simulink model "MMC_Rectifier_NLM_2018"  (R2023b)
settings: Solver=ode23t  StartTime=0.0  StopTime=3  RelTol=1e-3
libraries: spsIGBTDiodeLib x216, spsSeriesRLCBranchLib x117, spsVoltageMeasurementLib x110, spsCurrentMeasurementLib x7, slpidlib x6, spsThreePhaseVIMeasurementLib x2, spsGroundLib x1, spsPower3phInstantaneousLib x1, spsThreePhaseProgrammableVoltageSourceLib x1, spsThreePhaseSeriesRLCBranchLib x1, spspowerguiLib x1
(part 2 of 5)

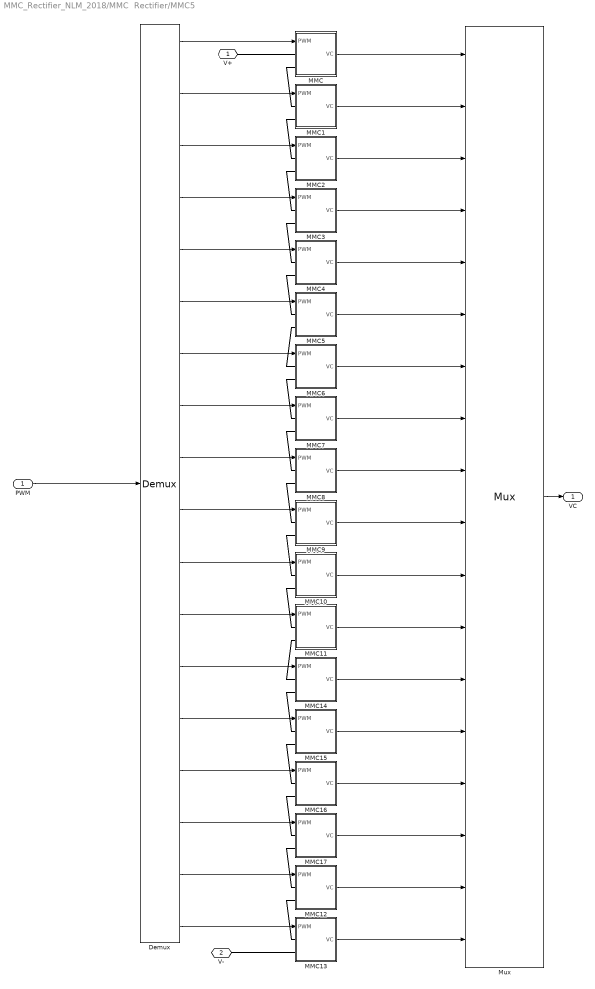
== system MMC_Rectifier_NLM_2018/MMC  Rectifier/MMC5 ==
  PWM : Inport
  Demux : Demux  Outputs=18
  MMC : Subsystem
  MMC1 : Subsystem
  MMC10 : Subsystem
  MMC11 : Subsystem
  MMC12 : Subsystem
  MMC13 : Subsystem
  MMC14 : Subsystem
  MMC15 : Subsystem
  MMC16 : Subsystem
  MMC17 : Subsystem
  MMC2 : Subsystem
  MMC3 : Subsystem
  MMC4 : Subsystem
  MMC5 : Subsystem
  MMC6 : Subsystem
  MMC7 : Subsystem
  MMC8 : Subsystem
  MMC9 : Subsystem
  Mux : Mux  Inputs=18
  V+ : PMIOPort  Side=Left
  V- : PMIOPort  Port=2  Side=Left
  VC : Outport
  wires:
  PWM/1 -> Demux/1
  Demux/18 -> MMC13/1(PWM)
  Demux/17 -> MMC12/1(PWM)
  Demux/16 -> MMC17/1(PWM)
  Demux/15 -> MMC16/1(PWM)
  Demux/14 -> MMC15/1(PWM)
  Demux/13 -> MMC14/1(PWM)
  Demux/12 -> MMC11/1(PWM)
  Demux/11 -> MMC10/1(PWM)
  Demux/10 -> MMC9/1(PWM)
  Demux/9 -> MMC8/1(PWM)
  Demux/8 -> MMC7/1(PWM)
  Demux/7 -> MMC6/1(PWM)
  Demux/6 -> MMC5/1(PWM)
  Demux/5 -> MMC4/1(PWM)
  Demux/4 -> MMC3/1(PWM)
  Demux/3 -> MMC2/1(PWM)
  Demux/2 -> MMC1/1(PWM)
  Demux/1 -> MMC/1(PWM)
  Mux/1 -> VC/1
  MMC13/1(VC) -> Mux/18
  MMC12/1(VC) -> Mux/17
  MMC17/1(VC) -> Mux/16
  MMC16/1(VC) -> Mux/15
  MMC15/1(VC) -> Mux/14
  MMC14/1(VC) -> Mux/13
  MMC11/1(VC) -> Mux/12
  MMC10/1(VC) -> Mux/11
  MMC9/1(VC) -> Mux/10
  MMC8/1(VC) -> Mux/9
  MMC7/1(VC) -> Mux/8
  MMC6/1(VC) -> Mux/7
  MMC5/1(VC) -> Mux/6
  MMC4/1(VC) -> Mux/5
  MMC3/1(VC) -> Mux/4
  MMC2/1(VC) -> Mux/3
  MMC1/1(VC) -> Mux/2
  MMC/1(VC) -> Mux/1
  connections:
  V+/RConn1 -- MMC/LConn1
  V-/RConn1 -- MMC13/LConn2
  MMC6/LConn1 -- MMC5/LConn2
  MMC14/LConn1 -- MMC11/LConn2
  MMC15/LConn2 -- MMC16/LConn1
  MMC17/LConn2 -- MMC12/LConn1
  MMC16/LConn2 -- MMC17/LConn1
  MMC14/LConn2 -- MMC15/LConn1
  MMC12/LConn2 -- MMC13/LConn1
  MMC10/LConn2 -- MMC11/LConn1
  MMC6/LConn2 -- MMC7/LConn1
  MMC7/LConn2 -- MMC8/LConn1
  MMC8/LConn2 -- MMC9/LConn1
  MMC9/LConn2 -- MMC10/LConn1
  MMC3/LConn2 -- MMC4/LConn1
  MMC2/LConn2 -- MMC3/LConn1
  MMC1/LConn2 -- MMC2/LConn1
  MMC/LConn2 -- MMC1/LConn1
  MMC4/LConn2 -- MMC5/LConn1

== system MMC_Rectifier_NLM_2018/坐标变换与锁相环/SOGI1 ==
  v : Inport
  Gain : Gain  Gain=sqrt(2)
  Gain1 : Gain  Gain=100*pi
  Gain2 : Gain  Gain=100*pi
  Integrator : Integrator
  Integrator1 : Integrator
  Sum : Sum  Inputs=|+-
  Sum1 : Sum  Inputs=|+-
  v' : Outport
  qv' : Outport  Port=2
  wires:
  Integrator1/1 -> qv'/1, Sum1/2
  Integrator/1 -> v'/1, Gain2/1, Sum/2
  Gain1/1 -> Integrator/1
  v/1 -> Sum/1
  Sum/1 -> Gain/1
  Sum1/1 -> Gain1/1
  Gain/1 -> Sum1/1
  Gain2/1 -> Integrator1/1

== system MMC_Rectifier_NLM_2018/坐标变换与锁相环/SOGI2 ==
  v : Inport
  Gain : Gain  Gain=sqrt(2)
  Gain1 : Gain  Gain=100*pi
  Gain2 : Gain  Gain=100*pi
  Integrator : Integrator
  Integrator1 : Integrator
  Sum : Sum  Inputs=|+-
  Sum1 : Sum  Inputs=|+-
  v' : Outport
  qv' : Outport  Port=2
  wires:
  Gain2/1 -> Integrator1/1
  Gain/1 -> Sum1/1
  Sum1/1 -> Gain1/1
  Sum/1 -> Gain/1
  v/1 -> Sum/1
  Gain1/1 -> Integrator/1
  Integrator/1 -> Sum/2, Gain2/1, v'/1
  Integrator1/1 -> Sum1/2, qv'/1

== system MMC_Rectifier_NLM_2018/子模块投入个数/Subsystem ==
  VA : Inport
  HLA : Inport  Port=2
  Constant2 : Constant  Value=N/2
  Constant3 : Constant  Value=1400
  Product : Product  Inputs=*/
  Round : Rounding  Operator=round
  Sum : Sum  Inputs=|+-
  Sum1 : Sum  Inputs=|++
  NAP : Outport
  wires:
  VA/1 -> Sum1/1
  HLA/1 -> Sum1/2
  Round/1 -> Sum/2
  Sum1/1 -> Product/1
  Constant2/1 -> Sum/1
  Product/1 -> Round/1
  Constant3/1 -> Product/2
  Sum/1 -> NAP/1

== system MMC_Rectifier_NLM_2018/子模块投入个数/Subsystem1 ==
  VA : Inport
  HLA : Inport  Port=2
  Constant2 : Constant  Value=N/2
  Constant3 : Constant  Value=1400
  Product : Product  Inputs=*/
  Round : Rounding  Operator=round
  Sum : Sum  Inputs=|++
  Sum1 : Sum  Inputs=|+-
  NAL : Outport
  wires:
  Sum/1 -> NAL/1
  Constant3/1 -> Product/2
  Product/1 -> Round/1
  Constant2/1 -> Sum/1
  Sum1/1 -> Product/1
  Round/1 -> Sum/2
  HLA/1 -> Sum1/2
  VA/1 -> Sum1/1

== system MMC_Rectifier_NLM_2018/子模块投入个数/Subsystem2 ==
  VB : Inport
  HLB : Inport  Port=2
  Constant2 : Constant  Value=N/2
  Constant3 : Constant  Value=1400
  Product : Product  Inputs=*/
  Round : Rounding  Operator=round
  Sum : Sum  Inputs=|+-
  Sum1 : Sum  Inputs=|++
  NBP : Outport
  wires:
  VB/1 -> Sum1/1
  HLB/1 -> Sum1/2
  Round/1 -> Sum/2
  Sum1/1 -> Product/1
  Constant2/1 -> Sum/1
  Product/1 -> Round/1
  Constant3/1 -> Product/2
  Sum/1 -> NBP/1

== system MMC_Rectifier_NLM_2018/子模块投入个数/Subsystem3 ==
  VB : Inport
  HLB : Inport  Port=2
  Constant2 : Constant  Value=N/2
  Constant3 : Constant  Value=1400
  Product : Product  Inputs=*/
  Round : Rounding  Operator=round
  Sum : Sum  Inputs=|++
  Sum1 : Sum  Inputs=|+-
  NBL : Outport
  wires:
  Sum/1 -> NBL/1
  Constant3/1 -> Product/2
  Product/1 -> Round/1
  Constant2/1 -> Sum/1
  Sum1/1 -> Product/1
  Round/1 -> Sum/2
  HLB/1 -> Sum1/2
  VB/1 -> Sum1/1

== system MMC_Rectifier_NLM_2018/子模块投入个数/Subsystem4 ==
  VC : Inport
  HLC : Inport  Port=2
  Constant2 : Constant  Value=N/2
  Constant3 : Constant  Value=1400
  Product : Product  Inputs=*/
  Round : Rounding  Operator=round
  Sum : Sum  Inputs=|+-
  Sum1 : Sum  Inputs=|++
  NCP : Outport
  wires:
  VC/1 -> Sum1/1
  HLC/1 -> Sum1/2
  Round/1 -> Sum/2
  Sum1/1 -> Product/1
  Constant2/1 -> Sum/1
  Product/1 -> Round/1
  Constant3/1 -> Product/2
  Sum/1 -> NCP/1

== system MMC_Rectifier_NLM_2018/子模块投入个数/Subsystem5 ==
  VC : Inport
  HLC : Inport  Port=2
  Constant2 : Constant  Value=N/2
  Constant3 : Constant  Value=1400
  Product : Product  Inputs=*/
  Round : Rounding  Operator=round
  Sum : Sum  Inputs=|++
  Sum1 : Sum  Inputs=|+-
  NCL : Outport
  wires:
  Sum/1 -> NCL/1
  Constant3/1 -> Product/2
  Product/1 -> Round/1
  Constant2/1 -> Sum/1
  Sum1/1 -> Product/1
  Round/1 -> Sum/2
  HLC/1 -> Sum1/2
  VC/1 -> Sum1/1

== system MMC_Rectifier_NLM_2018/MMC  Rectifier/MMC/MMC ==
  PWM : Inport
  IGBT/Diode : spsIGBTDiodeLib/IGBT//Diode  Ron=1e-3  Rs=1e5  Cs=inf  Measurements=off
  IGBT/Diode1 : spsIGBTDiodeLib/IGBT//Diode  Ron=1e-3  Rs=1e5  Cs=inf  Measurements=off
  Logical Operator : Logic  Inputs=1  AllPortsSameDT=off  OutDataTypeStr=boolean
  Logical Operator1 : Logic  Operator=NOT  Inputs=1  AllPortsSameDT=off  OutDataTypeStr=boolean
  Series RLC Branch : spsSeriesRLCBranchLib/Series RLC Branch  LConnTagsString=__new0  RConnTagsString=__new0  BranchType=C  Resistance=1  Inductance=1e-3  SetiL0=off  InitialCurrent=0  Capacitance=C0  Setx0=on  InitialVoltage=V0  Measurements=None
  Voltage Measurement : spsVoltageMeasurementLib/Voltage Measurement  PhasorSimulation=off  OutputType=Complex  PSBequivalent=0
  V+ : PMIOPort  Side=Left
  V- : PMIOPort  Port=2  Side=Left
  VC : Outport
  wires:
  PWM/1 -> Logical Operator1/1, Logical Operator/1
  Logical Operator/1 -> IGBT/Diode/1
  Voltage Measurement/1 -> VC/1
  Logical Operator1/1 -> IGBT/Diode1/1
  connections:
  Series RLC Branch/RConn1 -- Voltage Measurement/LConn2 -- V-/RConn1 -- IGBT/Diode1/RConn1
  IGBT/Diode1/LConn1 -- V+/RConn1 -- IGBT/Diode/RConn1
  Series RLC Branch/LConn1 -- Voltage Measurement/LConn1 -- IGBT/Diode/LConn1

== system MMC_Rectifier_NLM_2018/MMC  Rectifier/MMC/MMC1 ==
  PWM : Inport
  IGBT/Diode : spsIGBTDiodeLib/IGBT//Diode  Ron=1e-3  Rs=1e5  Cs=inf  Measurements=off
  IGBT/Diode1 : spsIGBTDiodeLib/IGBT//Diode  Ron=1e-3  Rs=1e5  Cs=inf  Measurements=off
  Logical Operator : Logic  Inputs=1  AllPortsSameDT=off  OutDataTypeStr=boolean
  Logical Operator1 : Logic  Operator=NOT  Inputs=1  AllPortsSameDT=off  OutDataTypeStr=boolean
  Series RLC Branch : spsSeriesRLCBranchLib/Series RLC Branch  LConnTagsString=__new0  RConnTagsString=__new0  BranchType=C  Resistance=1  Inductance=1e-3  SetiL0=off  InitialCurrent=0  Capacitance=C0  Setx0=on  InitialVoltage=V0  Measurements=None
  Voltage Measurement : spsVoltageMeasurementLib/Voltage Measurement  PhasorSimulation=off  OutputType=Complex  PSBequivalent=0
  V+ : PMIOPort  Side=Left
  V- : PMIOPort  Port=2  Side=Left
  VC : Outport
  wires:
  Logical Operator1/1 -> IGBT/Diode1/1
  Voltage Measurement/1 -> VC/1
  Logical Operator/1 -> IGBT/Diode/1
  PWM/1 -> Logical Operator/1, Logical Operator1/1
  connections:
  Voltage Measurement/LConn1 -- Series RLC Branch/LConn1 -- IGBT/Diode/LConn1
  V+/RConn1 -- IGBT/Diode1/LConn1 -- IGBT/Diode/RConn1
  V-/RConn1 -- IGBT/Diode1/RConn1 -- Series RLC Branch/RConn1 -- Voltage Measurement/LConn2

== system MMC_Rectifier_NLM_2018/MMC  Rectifier/MMC/MMC10 ==
  PWM : Inport
  IGBT/Diode : spsIGBTDiodeLib/IGBT//Diode  Ron=1e-3  Rs=1e5  Cs=inf  Measurements=off
  IGBT/Diode1 : spsIGBTDiodeLib/IGBT//Diode  Ron=1e-3  Rs=1e5  Cs=inf  Measurements=off
  Logical Operator : Logic  Inputs=1  AllPortsSameDT=off  OutDataTypeStr=boolean
  Logical Operator1 : Logic  Operator=NOT  Inputs=1  AllPortsSameDT=off  OutDataTypeStr=boolean
  Series RLC Branch : spsSeriesRLCBranchLib/Series RLC Branch  LConnTagsString=__new0  RConnTagsString=__new0  BranchType=C  Resistance=1  Inductance=1e-3  SetiL0=off  InitialCurrent=0  Capacitance=C0  Setx0=on  InitialVoltage=V0  Measurements=None
  Voltage Measurement : spsVoltageMeasurementLib/Voltage Measurement  PhasorSimulation=off  OutputType=Complex  PSBequivalent=0
  V+ : PMIOPort  Side=Left
  V- : PMIOPort  Port=2  Side=Left
  VC : Outport
  wires:
  Logical Operator1/1 -> IGBT/Diode1/1
  Voltage Measurement/1 -> VC/1
  Logical Operator/1 -> IGBT/Diode/1
  PWM/1 -> Logical Operator/1, Logical Operator1/1
  connections:
  Voltage Measurement/LConn1 -- Series RLC Branch/LConn1 -- IGBT/Diode/LConn1
  V+/RConn1 -- IGBT/Diode1/LConn1 -- IGBT/Diode/RConn1
  V-/RConn1 -- IGBT/Diode1/RConn1 -- Series RLC Branch/RConn1 -- Voltage Measurement/LConn2

== system MMC_Rectifier_NLM_2018/MMC  Rectifier/MMC/MMC11 ==
  PWM : Inport
  IGBT/Diode : spsIGBTDiodeLib/IGBT//Diode  Ron=1e-3  Rs=1e5  Cs=inf  Measurements=off
  IGBT/Diode1 : spsIGBTDiodeLib/IGBT//Diode  Ron=1e-3  Rs=1e5  Cs=inf  Measurements=off
  Logical Operator : Logic  Inputs=1  AllPortsSameDT=off  OutDataTypeStr=boolean
  Logical Operator1 : Logic  Operator=NOT  Inputs=1  AllPortsSameDT=off  OutDataTypeStr=boolean
  Series RLC Branch : spsSeriesRLCBranchLib/Series RLC Branch  LConnTagsString=__new0  RConnTagsString=__new0  BranchType=C  Resistance=1  Inductance=1e-3  SetiL0=off  InitialCurrent=0  Capacitance=C0  Setx0=on  InitialVoltage=V0  Measurements=None
  Voltage Measurement : spsVoltageMeasurementLib/Voltage Measurement  PhasorSimulation=off  OutputType=Complex  PSBequivalent=0
  V+ : PMIOPort  Side=Left
  V- : PMIOPort  Port=2  Side=Left
  VC : Outport
  wires:
  PWM/1 -> Logical Operator1/1, Logical Operator/1
  Logical Operator/1 -> IGBT/Diode/1
  Voltage Measurement/1 -> VC/1
  Logical Operator1/1 -> IGBT/Diode1/1
  connections:
  Voltage Measurement/LConn2 -- Series RLC Branch/RConn1 -- IGBT/Diode1/RConn1 -- V-/RConn1
  IGBT/Diode/RConn1 -- IGBT/Diode1/LConn1 -- V+/RConn1
  IGBT/Diode/LConn1 -- Series RLC Branch/LConn1 -- Voltage Measurement/LConn1

== system MMC_Rectifier_NLM_2018/MMC  Rectifier/MMC/MMC12 ==
  PWM : Inport
  IGBT/Diode : spsIGBTDiodeLib/IGBT//Diode  Ron=1e-3  Rs=1e5  Cs=inf  Measurements=off
  IGBT/Diode1 : spsIGBTDiodeLib/IGBT//Diode  Ron=1e-3  Rs=1e5  Cs=inf  Measurements=off
  Logical Operator : Logic  Inputs=1  AllPortsSameDT=off  OutDataTypeStr=boolean
  Logical Operator1 : Logic  Operator=NOT  Inputs=1  AllPortsSameDT=off  OutDataTypeStr=boolean
  Series RLC Branch : spsSeriesRLCBranchLib/Series RLC Branch  LConnTagsString=__new0  RConnTagsString=__new0  BranchType=C  Resistance=1  Inductance=1e-3  SetiL0=off  InitialCurrent=0  Capacitance=C0  Setx0=on  InitialVoltage=V0  Measurements=None
  Voltage Measurement : spsVoltageMeasurementLib/Voltage Measurement  PhasorSimulation=off  OutputType=Complex  PSBequivalent=0
  V+ : PMIOPort  Side=Left
  V- : PMIOPort  Port=2  Side=Left
  VC : Outport
  wires:
  PWM/1 -> Logical Operator1/1, Logical Operator/1
  Logical Operator/1 -> IGBT/Diode/1
  Voltage Measurement/1 -> VC/1
  Logical Operator1/1 -> IGBT/Diode1/1
  connections:
  Voltage Measurement/LConn2 -- Series RLC Branch/RConn1 -- IGBT/Diode1/RConn1 -- V-/RConn1
  IGBT/Diode/RConn1 -- IGBT/Diode1/LConn1 -- V+/RConn1
  IGBT/Diode/LConn1 -- Series RLC Branch/LConn1 -- Voltage Measurement/LConn1

== system MMC_Rectifier_NLM_2018/MMC  Rectifier/MMC/MMC13 ==
  PWM : Inport
  IGBT/Diode : spsIGBTDiodeLib/IGBT//Diode  Ron=1e-3  Rs=1e5  Cs=inf  Measurements=off
  IGBT/Diode1 : spsIGBTDiodeLib/IGBT//Diode  Ron=1e-3  Rs=1e5  Cs=inf  Measurements=off
  Logical Operator : Logic  Inputs=1  AllPortsSameDT=off  OutDataTypeStr=boolean
  Logical Operator1 : Logic  Operator=NOT  Inputs=1  AllPortsSameDT=off  OutDataTypeStr=boolean
  Series RLC Branch : spsSeriesRLCBranchLib/Series RLC Branch  LConnTagsString=__new0  RConnTagsString=__new0  BranchType=C  Resistance=1  Inductance=1e-3  SetiL0=off  InitialCurrent=0  Capacitance=C0  Setx0=on  InitialVoltage=V0  Measurements=None
  Voltage Measurement : spsVoltageMeasurementLib/Voltage Measurement  PhasorSimulation=off  OutputType=Complex  PSBequivalent=0
  V+ : PMIOPort  Side=Left
  V- : PMIOPort  Port=2  Side=Left
  VC : Outport
  wires:
  Logical Operator1/1 -> IGBT/Diode1/1
  Voltage Measurement/1 -> VC/1
  Logical Operator/1 -> IGBT/Diode/1
  PWM/1 -> Logical Operator/1, Logical Operator1/1
  connections:
  Voltage Measurement/LConn1 -- Series RLC Branch/LConn1 -- IGBT/Diode/LConn1
  V+/RConn1 -- IGBT/Diode1/LConn1 -- IGBT/Diode/RConn1
  V-/RConn1 -- IGBT/Diode1/RConn1 -- Series RLC Branch/RConn1 -- Voltage Measurement/LConn2

== system MMC_Rectifier_NLM_2018/MMC  Rectifier/MMC/MMC14 ==
  PWM : Inport
  IGBT/Diode : spsIGBTDiodeLib/IGBT//Diode  Ron=1e-3  Rs=1e5  Cs=inf  Measurements=off
  IGBT/Diode1 : spsIGBTDiodeLib/IGBT//Diode  Ron=1e-3  Rs=1e5  Cs=inf  Measurements=off
  Logical Operator : Logic  Inputs=1  AllPortsSameDT=off  OutDataTypeStr=boolean
  Logical Operator1 : Logic  Operator=NOT  Inputs=1  AllPortsSameDT=off  OutDataTypeStr=boolean
  Series RLC Branch : spsSeriesRLCBranchLib/Series RLC Branch  LConnTagsString=__new0  RConnTagsString=__new0  BranchType=C  Resistance=1  Inductance=1e-3  SetiL0=off  InitialCurrent=0  Capacitance=C0  Setx0=on  InitialVoltage=V0  Measurements=None
  Voltage Measurement : spsVoltageMeasurementLib/Voltage Measurement  PhasorSimulation=off  OutputType=Complex  PSBequivalent=0
  V+ : PMIOPort  Side=Left
  V- : PMIOPort  Port=2  Side=Left
  VC : Outport
  wires:
  PWM/1 -> Logical Operator1/1, Logical Operator/1
  Logical Operator/1 -> IGBT/Diode/1
  Voltage Measurement/1 -> VC/1
  Logical Operator1/1 -> IGBT/Diode1/1
  connections:
  Series RLC Branch/RConn1 -- Voltage Measurement/LConn2 -- V-/RConn1 -- IGBT/Diode1/RConn1
  IGBT/Diode1/LConn1 -- V+/RConn1 -- IGBT/Diode/RConn1
  Series RLC Branch/LConn1 -- Voltage Measurement/LConn1 -- IGBT/Diode/LConn1

== system MMC_Rectifier_NLM_2018/MMC  Rectifier/MMC/MMC15 ==
  PWM : Inport
  IGBT/Diode : spsIGBTDiodeLib/IGBT//Diode  Ron=1e-3  Rs=1e5  Cs=inf  Measurements=off
  IGBT/Diode1 : spsIGBTDiodeLib/IGBT//Diode  Ron=1e-3  Rs=1e5  Cs=inf  Measurements=off
  Logical Operator : Logic  Inputs=1  AllPortsSameDT=off  OutDataTypeStr=boolean
  Logical Operator1 : Logic  Operator=NOT  Inputs=1  AllPortsSameDT=off  OutDataTypeStr=boolean
  Series RLC Branch : spsSeriesRLCBranchLib/Series RLC Branch  LConnTagsString=__new0  RConnTagsString=__new0  BranchType=C  Resistance=1  Inductance=1e-3  SetiL0=off  InitialCurrent=0  Capacitance=C0  Setx0=on  InitialVoltage=V0  Measurements=None
  Voltage Measurement : spsVoltageMeasurementLib/Voltage Measurement  PhasorSimulation=off  OutputType=Complex  PSBequivalent=0
  V+ : PMIOPort  Side=Left
  V- : PMIOPort  Port=2  Side=Left
  VC : Outport
  wires:
  Logical Operator1/1 -> IGBT/Diode1/1
  Voltage Measurement/1 -> VC/1
  Logical Operator/1 -> IGBT/Diode/1
  PWM/1 -> Logical Operator/1, Logical Operator1/1
  connections:
  Voltage Measurement/LConn1 -- Series RLC Branch/LConn1 -- IGBT/Diode/LConn1
  V+/RConn1 -- IGBT/Diode1/LConn1 -- IGBT/Diode/RConn1
  V-/RConn1 -- IGBT/Diode1/RConn1 -- Series RLC Branch/RConn1 -- Voltage Measurement/LConn2

== system MMC_Rectifier_NLM_2018/MMC  Rectifier/MMC/MMC16 ==
  PWM : Inport
  IGBT/Diode : spsIGBTDiodeLib/IGBT//Diode  Ron=1e-3  Rs=1e5  Cs=inf  Measurements=off
  IGBT/Diode1 : spsIGBTDiodeLib/IGBT//Diode  Ron=1e-3  Rs=1e5  Cs=inf  Measurements=off
  Logical Operator : Logic  Inputs=1  AllPortsSameDT=off  OutDataTypeStr=boolean
  Logical Operator1 : Logic  Operator=NOT  Inputs=1  AllPortsSameDT=off  OutDataTypeStr=boolean
  Series RLC Branch : spsSeriesRLCBranchLib/Series RLC Branch  LConnTagsString=__new0  RConnTagsString=__new0  BranchType=C  Resistance=1  Inductance=1e-3  SetiL0=off  InitialCurrent=0  Capacitance=C0  Setx0=on  InitialVoltage=V0  Measurements=None
  Voltage Measurement : spsVoltageMeasurementLib/Voltage Measurement  PhasorSimulation=off  OutputType=Complex  PSBequivalent=0
  V+ : PMIOPort  Side=Left
  V- : PMIOPort  Port=2  Side=Left
  VC : Outport
  wires:
  Logical Operator1/1 -> IGBT/Diode1/1
  Voltage Measurement/1 -> VC/1
  Logical Operator/1 -> IGBT/Diode/1
  PWM/1 -> Logical Operator/1, Logical Operator1/1
  connections:
  Voltage Measurement/LConn1 -- Series RLC Branch/LConn1 -- IGBT/Diode/LConn1
  V+/RConn1 -- IGBT/Diode1/LConn1 -- IGBT/Diode/RConn1
  V-/RConn1 -- IGBT/Diode1/RConn1 -- Series RLC Branch/RConn1 -- Voltage Measurement/LConn2

== system MMC_Rectifier_NLM_2018/MMC  Rectifier/MMC/MMC17 ==
  PWM : Inport
  IGBT/Diode : spsIGBTDiodeLib/IGBT//Diode  Ron=1e-3  Rs=1e5  Cs=inf  Measurements=off
  IGBT/Diode1 : spsIGBTDiodeLib/IGBT//Diode  Ron=1e-3  Rs=1e5  Cs=inf  Measurements=off
  Logical Operator : Logic  Inputs=1  AllPortsSameDT=off  OutDataTypeStr=boolean
  Logical Operator1 : Logic  Operator=NOT  Inputs=1  AllPortsSameDT=off  OutDataTypeStr=boolean
  Series RLC Branch : spsSeriesRLCBranchLib/Series RLC Branch  LConnTagsString=__new0  RConnTagsString=__new0  BranchType=C  Resistance=1  Inductance=1e-3  SetiL0=off  InitialCurrent=0  Capacitance=C0  Setx0=on  InitialVoltage=V0  Measurements=None
  Voltage Measurement : spsVoltageMeasurementLib/Voltage Measurement  PhasorSimulation=off  OutputType=Complex  PSBequivalent=0
  V+ : PMIOPort  Side=Left
  V- : PMIOPort  Port=2  Side=Left
  VC : Outport
  wires:
  PWM/1 -> Logical Operator1/1, Logical Operator/1
  Logical Operator/1 -> IGBT/Diode/1
  Voltage Measurement/1 -> VC/1
  Logical Operator1/1 -> IGBT/Diode1/1
  connections:
  Voltage Measurement/LConn2 -- Series RLC Branch/RConn1 -- IGBT/Diode1/RConn1 -- V-/RConn1
  IGBT/Diode/RConn1 -- IGBT/Diode1/LConn1 -- V+/RConn1
  IGBT/Diode/LConn1 -- Series RLC Branch/LConn1 -- Voltage Measurement/LConn1

== system MMC_Rectifier_NLM_2018/MMC  Rectifier/MMC/MMC2 ==
  PWM : Inport
  IGBT/Diode : spsIGBTDiodeLib/IGBT//Diode  Ron=1e-3  Rs=1e5  Cs=inf  Measurements=off
  IGBT/Diode1 : spsIGBTDiodeLib/IGBT//Diode  Ron=1e-3  Rs=1e5  Cs=inf  Measurements=off
  Logical Operator : Logic  Inputs=1  AllPortsSameDT=off  OutDataTypeStr=boolean
  Logical Operator1 : Logic  Operator=NOT  Inputs=1  AllPortsSameDT=off  OutDataTypeStr=boolean
  Series RLC Branch : spsSeriesRLCBranchLib/Series RLC Branch  LConnTagsString=__new0  RConnTagsString=__new0  BranchType=C  Resistance=1  Inductance=1e-3  SetiL0=off  InitialCurrent=0  Capacitance=C0  Setx0=on  InitialVoltage=V0  Measurements=None
  Voltage Measurement : spsVoltageMeasurementLib/Voltage Measurement  PhasorSimulation=off  OutputType=Complex  PSBequivalent=0
  V+ : PMIOPort  Side=Left
  V- : PMIOPort  Port=2  Side=Left
  VC : Outport
  wires:
  Logical Operator1/1 -> IGBT/Diode1/1
  Voltage Measurement/1 -> VC/1
  Logical Operator/1 -> IGBT/Diode/1
  PWM/1 -> Logical Operator/1, Logical Operator1/1
  connections:
  Voltage Measurement/LConn1 -- Series RLC Branch/LConn1 -- IGBT/Diode/LConn1
  V+/RConn1 -- IGBT/Diode1/LConn1 -- IGBT/Diode/RConn1
  V-/RConn1 -- IGBT/Diode1/RConn1 -- Series RLC Branch/RConn1 -- Voltage Measurement/LConn2

== system MMC_Rectifier_NLM_2018/MMC  Rectifier/MMC/MMC3 ==
  PWM : Inport
  IGBT/Diode : spsIGBTDiodeLib/IGBT//Diode  Ron=1e-3  Rs=1e5  Cs=inf  Measurements=off
  IGBT/Diode1 : spsIGBTDiodeLib/IGBT//Diode  Ron=1e-3  Rs=1e5  Cs=inf  Measurements=off
  Logical Operator : Logic  Inputs=1  AllPortsSameDT=off  OutDataTypeStr=boolean
  Logical Operator1 : Logic  Operator=NOT  Inputs=1  AllPortsSameDT=off  OutDataTypeStr=boolean
  Series RLC Branch : spsSeriesRLCBranchLib/Series RLC Branch  LConnTagsString=__new0  RConnTagsString=__new0  BranchType=C  Resistance=1  Inductance=1e-3  SetiL0=off  InitialCurrent=0  Capacitance=C0  Setx0=on  InitialVoltage=V0  Measurements=None
  Voltage Measurement : spsVoltageMeasurementLib/Voltage Measurement  PhasorSimulation=off  OutputType=Complex  PSBequivalent=0
  V+ : PMIOPort  Side=Left
  V- : PMIOPort  Port=2  Side=Left
  VC : Outport
  wires:
  PWM/1 -> Logical Operator1/1, Logical Operator/1
  Logical Operator/1 -> IGBT/Diode/1
  Voltage Measurement/1 -> VC/1
  Logical Operator1/1 -> IGBT/Diode1/1
  connections:
  Voltage Measurement/LConn2 -- Series RLC Branch/RConn1 -- IGBT/Diode1/RConn1 -- V-/RConn1
  IGBT/Diode/RConn1 -- IGBT/Diode1/LConn1 -- V+/RConn1
  IGBT/Diode/LConn1 -- Series RLC Branch/LConn1 -- Voltage Measurement/LConn1

== system MMC_Rectifier_NLM_2018/MMC  Rectifier/MMC/MMC4 ==
  PWM : Inport
  IGBT/Diode : spsIGBTDiodeLib/IGBT//Diode  Ron=1e-3  Rs=1e5  Cs=inf  Measurements=off
  IGBT/Diode1 : spsIGBTDiodeLib/IGBT//Diode  Ron=1e-3  Rs=1e5  Cs=inf  Measurements=off
  Logical Operator : Logic  Inputs=1  AllPortsSameDT=off  OutDataTypeStr=boolean
  Logical Operator1 : Logic  Operator=NOT  Inputs=1  AllPortsSameDT=off  OutDataTypeStr=boolean
  Series RLC Branch : spsSeriesRLCBranchLib/Series RLC Branch  LConnTagsString=__new0  RConnTagsString=__new0  BranchType=C  Resistance=1  Inductance=1e-3  SetiL0=off  InitialCurrent=0  Capacitance=C0  Setx0=on  InitialVoltage=V0  Measurements=None
  Voltage Measurement : spsVoltageMeasurementLib/Voltage Measurement  PhasorSimulation=off  OutputType=Complex  PSBequivalent=0
  V+ : PMIOPort  Side=Left
  V- : PMIOPort  Port=2  Side=Left
  VC : Outport
  wires:
  PWM/1 -> Logical Operator1/1, Logical Operator/1
  Logical Operator/1 -> IGBT/Diode/1
  Voltage Measurement/1 -> VC/1
  Logical Operator1/1 -> IGBT/Diode1/1
  connections:
  Voltage Measurement/LConn2 -- Series RLC Branch/RConn1 -- IGBT/Diode1/RConn1 -- V-/RConn1
  IGBT/Diode/RConn1 -- IGBT/Diode1/LConn1 -- V+/RConn1
  IGBT/Diode/LConn1 -- Series RLC Branch/LConn1 -- Voltage Measurement/LConn1

== system MMC_Rectifier_NLM_2018/MMC  Rectifier/MMC/MMC5 ==
  PWM : Inport
  IGBT/Diode : spsIGBTDiodeLib/IGBT//Diode  Ron=1e-3  Rs=1e5  Cs=inf  Measurements=off
  IGBT/Diode1 : spsIGBTDiodeLib/IGBT//Diode  Ron=1e-3  Rs=1e5  Cs=inf  Measurements=off
  Logical Operator : Logic  Inputs=1  AllPortsSameDT=off  OutDataTypeStr=boolean
  Logical Operator1 : Logic  Operator=NOT  Inputs=1  AllPortsSameDT=off  OutDataTypeStr=boolean
  Series RLC Branch : spsSeriesRLCBranchLib/Series RLC Branch  LConnTagsString=__new0  RConnTagsString=__new0  BranchType=C  Resistance=1  Inductance=1e-3  SetiL0=off  InitialCurrent=0  Capacitance=C0  Setx0=on  InitialVoltage=V0  Measurements=None
  Voltage Measurement : spsVoltageMeasurementLib/Voltage Measurement  PhasorSimulation=off  OutputType=Complex  PSBequivalent=0
  V+ : PMIOPort  Side=Left
  V- : PMIOPort  Port=2  Side=Left
  VC : Outport
  wires:
  Logical Operator1/1 -> IGBT/Diode1/1
  Voltage Measurement/1 -> VC/1
  Logical Operator/1 -> IGBT/Diode/1
  PWM/1 -> Logical Operator/1, Logical Operator1/1
  connections:
  Voltage Measurement/LConn1 -- Series RLC Branch/LConn1 -- IGBT/Diode/LConn1
  V+/RConn1 -- IGBT/Diode1/LConn1 -- IGBT/Diode/RConn1
  V-/RConn1 -- IGBT/Diode1/RConn1 -- Series RLC Branch/RConn1 -- Voltage Measurement/LConn2

== system MMC_Rectifier_NLM_2018/MMC  Rectifier/MMC/MMC6 ==
  PWM : Inport
  IGBT/Diode : spsIGBTDiodeLib/IGBT//Diode  Ron=1e-3  Rs=1e5  Cs=inf  Measurements=off
  IGBT/Diode1 : spsIGBTDiodeLib/IGBT//Diode  Ron=1e-3  Rs=1e5  Cs=inf  Measurements=off
  Logical Operator : Logic  Inputs=1  AllPortsSameDT=off  OutDataTypeStr=boolean
  Logical Operator1 : Logic  Operator=NOT  Inputs=1  AllPortsSameDT=off  OutDataTypeStr=boolean
  Series RLC Branch : spsSeriesRLCBranchLib/Series RLC Branch  LConnTagsString=__new0  RConnTagsString=__new0  BranchType=C  Resistance=1  Inductance=1e-3  SetiL0=off  InitialCurrent=0  Capacitance=C0  Setx0=on  InitialVoltage=V0  Measurements=None
  Voltage Measurement : spsVoltageMeasurementLib/Voltage Measurement  PhasorSimulation=off  OutputType=Complex  PSBequivalent=0
  V+ : PMIOPort  Side=Left
  V- : PMIOPort  Port=2  Side=Left
  VC : Outport
  wires:
  Logical Operator1/1 -> IGBT/Diode1/1
  Voltage Measurement/1 -> VC/1
  Logical Operator/1 -> IGBT/Diode/1
  PWM/1 -> Logical Operator/1, Logical Operator1/1
  connections:
  IGBT/Diode/LConn1 -- Voltage Measurement/LConn1 -- Series RLC Branch/LConn1
  IGBT/Diode/RConn1 -- V+/RConn1 -- IGBT/Diode1/LConn1
  IGBT/Diode1/RConn1 -- V-/RConn1 -- Voltage Measurement/LConn2 -- Series RLC Branch/RConn1

== system MMC_Rectifier_NLM_2018/MMC  Rectifier/MMC/MMC7 ==
  PWM : Inport
  IGBT/Diode : spsIGBTDiodeLib/IGBT//Diode  Ron=1e-3  Rs=1e5  Cs=inf  Measurements=off
  IGBT/Diode1 : spsIGBTDiodeLib/IGBT//Diode  Ron=1e-3  Rs=1e5  Cs=inf  Measurements=off
  Logical Operator : Logic  Inputs=1  AllPortsSameDT=off  OutDataTypeStr=boolean
  Logical Operator1 : Logic  Operator=NOT  Inputs=1  AllPortsSameDT=off  OutDataTypeStr=boolean
  Series RLC Branch : spsSeriesRLCBranchLib/Series RLC Branch  LConnTagsString=__new0  RConnTagsString=__new0  BranchType=C  Resistance=1  Inductance=1e-3  SetiL0=off  InitialCurrent=0  Capacitance=C0  Setx0=on  InitialVoltage=V0  Measurements=None
  Voltage Measurement : spsVoltageMeasurementLib/Voltage Measurement  PhasorSimulation=off  OutputType=Complex  PSBequivalent=0
  V+ : PMIOPort  Side=Left
  V- : PMIOPort  Port=2  Side=Left
  VC : Outport
  wires:
  PWM/1 -> Logical Operator1/1, Logical Operator/1
  Logical Operator/1 -> IGBT/Diode/1
  Voltage Measurement/1 -> VC/1
  Logical Operator1/1 -> IGBT/Diode1/1
  connections:
  Voltage Measurement/LConn2 -- Series RLC Branch/RConn1 -- IGBT/Diode1/RConn1 -- V-/RConn1
  IGBT/Diode/RConn1 -- IGBT/Diode1/LConn1 -- V+/RConn1
  IGBT/Diode/LConn1 -- Series RLC Branch/LConn1 -- Voltage Measurement/LConn1

== system MMC_Rectifier_NLM_2018/MMC  Rectifier/MMC/MMC8 ==
  PWM : Inport
  IGBT/Diode : spsIGBTDiodeLib/IGBT//Diode  Ron=1e-3  Rs=1e5  Cs=inf  Measurements=off
  IGBT/Diode1 : spsIGBTDiodeLib/IGBT//Diode  Ron=1e-3  Rs=1e5  Cs=inf  Measurements=off
  Logical Operator : Logic  Inputs=1  AllPortsSameDT=off  OutDataTypeStr=boolean
  Logical Operator1 : Logic  Operator=NOT  Inputs=1  AllPortsSameDT=off  OutDataTypeStr=boolean
  Series RLC Branch : spsSeriesRLCBranchLib/Series RLC Branch  LConnTagsString=__new0  RConnTagsString=__new0  BranchType=C  Resistance=1  Inductance=1e-3  SetiL0=off  InitialCurrent=0  Capacitance=C0  Setx0=on  InitialVoltage=V0  Measurements=None
  Voltage Measurement : spsVoltageMeasurementLib/Voltage Measurement  PhasorSimulation=off  OutputType=Complex  PSBequivalent=0
  V+ : PMIOPort  Side=Left
  V- : PMIOPort  Port=2  Side=Left
  VC : Outport
  wires:
  PWM/1 -> Logical Operator1/1, Logical Operator/1
  Logical Operator/1 -> IGBT/Diode/1
  Voltage Measurement/1 -> VC/1
  Logical Operator1/1 -> IGBT/Diode1/1
  connections:
  Voltage Measurement/LConn2 -- Series RLC Branch/RConn1 -- IGBT/Diode1/RConn1 -- V-/RConn1
  IGBT/Diode/RConn1 -- IGBT/Diode1/LConn1 -- V+/RConn1
  IGBT/Diode/LConn1 -- Series RLC Branch/LConn1 -- Voltage Measurement/LConn1

== system MMC_Rectifier_NLM_2018/MMC  Rectifier/MMC/MMC9 ==
  PWM : Inport
  IGBT/Diode : spsIGBTDiodeLib/IGBT//Diode  Ron=1e-3  Rs=1e5  Cs=inf  Measurements=off
  IGBT/Diode1 : spsIGBTDiodeLib/IGBT//Diode  Ron=1e-3  Rs=1e5  Cs=inf  Measurements=off
  Logical Operator : Logic  Inputs=1  AllPortsSameDT=off  OutDataTypeStr=boolean
  Logical Operator1 : Logic  Operator=NOT  Inputs=1  AllPortsSameDT=off  OutDataTypeStr=boolean
  Series RLC Branch : spsSeriesRLCBranchLib/Series RLC Branch  LConnTagsString=__new0  RConnTagsString=__new0  BranchType=C  Resistance=1  Inductance=1e-3  SetiL0=off  InitialCurrent=0  Capacitance=C0  Setx0=on  InitialVoltage=V0  Measurements=None
  Voltage Measurement : spsVoltageMeasurementLib/Voltage Measurement  PhasorSimulation=off  OutputType=Complex  PSBequivalent=0
  V+ : PMIOPort  Side=Left
  V- : PMIOPort  Port=2  Side=Left
  VC : Outport
  wires:
  Logical Operator1/1 -> IGBT/Diode1/1
  Voltage Measurement/1 -> VC/1
  Logical Operator/1 -> IGBT/Diode/1
  PWM/1 -> Logical Operator/1, Logical Operator1/1
  connections:
  Voltage Measurement/LConn1 -- Series RLC Branch/LConn1 -- IGBT/Diode/LConn1
  V+/RConn1 -- IGBT/Diode1/LConn1 -- IGBT/Diode/RConn1
  V-/RConn1 -- IGBT/Diode1/RConn1 -- Series RLC Branch/RConn1 -- Voltage Measurement/LConn2

== system MMC_Rectifier_NLM_2018/MMC  Rectifier/MMC1/MMC ==
  PWM : Inport
  IGBT/Diode : spsIGBTDiodeLib/IGBT//Diode  Ron=1e-3  Rs=1e5  Cs=inf  Measurements=off
  IGBT/Diode1 : spsIGBTDiodeLib/IGBT//Diode  Ron=1e-3  Rs=1e5  Cs=inf  Measurements=off
  Logical Operator : Logic  Inputs=1  AllPortsSameDT=off  OutDataTypeStr=boolean
  Logical Operator1 : Logic  Operator=NOT  Inputs=1  AllPortsSameDT=off  OutDataTypeStr=boolean
  Series RLC Branch : spsSeriesRLCBranchLib/Series RLC Branch  LConnTagsString=__new0  RConnTagsString=__new0  BranchType=C  Resistance=1  Inductance=1e-3  SetiL0=off  InitialCurrent=0  Capacitance=C0  Setx0=on  InitialVoltage=V0  Measurements=None
  Voltage Measurement : spsVoltageMeasurementLib/Voltage Measurement  PhasorSimulation=off  OutputType=Complex  PSBequivalent=0
  V+ : PMIOPort  Side=Left
  V- : PMIOPort  Port=2  Side=Left
  VC : Outport
  wires:
  Logical Operator1/1 -> IGBT/Diode1/1
  Voltage Measurement/1 -> VC/1
  Logical Operator/1 -> IGBT/Diode/1
  PWM/1 -> Logical Operator/1, Logical Operator1/1
  connections:
  IGBT/Diode/LConn1 -- Voltage Measurement/LConn1 -- Series RLC Branch/LConn1
  IGBT/Diode/RConn1 -- V+/RConn1 -- IGBT/Diode1/LConn1
  IGBT/Diode1/RConn1 -- V-/RConn1 -- Voltage Measurement/LConn2 -- Series RLC Branch/RConn1

== system MMC_Rectifier_NLM_2018/MMC  Rectifier/MMC1/MMC1 ==
  PWM : Inport
  IGBT/Diode : spsIGBTDiodeLib/IGBT//Diode  Ron=1e-3  Rs=1e5  Cs=inf  Measurements=off
  IGBT/Diode1 : spsIGBTDiodeLib/IGBT//Diode  Ron=1e-3  Rs=1e5  Cs=inf  Measurements=off
  Logical Operator : Logic  Inputs=1  AllPortsSameDT=off  OutDataTypeStr=boolean
  Logical Operator1 : Logic  Operator=NOT  Inputs=1  AllPortsSameDT=off  OutDataTypeStr=boolean
  Series RLC Branch : spsSeriesRLCBranchLib/Series RLC Branch  LConnTagsString=__new0  RConnTagsString=__new0  BranchType=C  Resistance=1  Inductance=1e-3  SetiL0=off  InitialCurrent=0  Capacitance=C0  Setx0=on  InitialVoltage=V0  Measurements=None
  Voltage Measurement : spsVoltageMeasurementLib/Voltage Measurement  PhasorSimulation=off  OutputType=Complex  PSBequivalent=0
  V+ : PMIOPort  Side=Left
  V- : PMIOPort  Port=2  Side=Left
  VC : Outport
  wires:
  PWM/1 -> Logical Operator1/1, Logical Operator/1
  Logical Operator/1 -> IGBT/Diode/1
  Voltage Measurement/1 -> VC/1
  Logical Operator1/1 -> IGBT/Diode1/1
  connections:
  Voltage Measurement/LConn2 -- Series RLC Branch/RConn1 -- IGBT/Diode1/RConn1 -- V-/RConn1
  IGBT/Diode/RConn1 -- IGBT/Diode1/LConn1 -- V+/RConn1
  IGBT/Diode/LConn1 -- Series RLC Branch/LConn1 -- Voltage Measurement/LConn1

== system MMC_Rectifier_NLM_2018/MMC  Rectifier/MMC1/MMC10 ==
  PWM : Inport
  IGBT/Diode : spsIGBTDiodeLib/IGBT//Diode  Ron=1e-3  Rs=1e5  Cs=inf  Measurements=off
  IGBT/Diode1 : spsIGBTDiodeLib/IGBT//Diode  Ron=1e-3  Rs=1e5  Cs=inf  Measurements=off
  Logical Operator : Logic  Inputs=1  AllPortsSameDT=off  OutDataTypeStr=boolean
  Logical Operator1 : Logic  Operator=NOT  Inputs=1  AllPortsSameDT=off  OutDataTypeStr=boolean
  Series RLC Branch : spsSeriesRLCBranchLib/Series RLC Branch  LConnTagsString=__new0  RConnTagsString=__new0  BranchType=C  Resistance=1  Inductance=1e-3  SetiL0=off  InitialCurrent=0  Capacitance=C0  Setx0=on  InitialVoltage=V0  Measurements=None
  Voltage Measurement : spsVoltageMeasurementLib/Voltage Measurement  PhasorSimulation=off  OutputType=Complex  PSBequivalent=0
  V+ : PMIOPort  Side=Left
  V- : PMIOPort  Port=2  Side=Left
  VC : Outport
  wires:
  PWM/1 -> Logical Operator1/1, Logical Operator/1
  Logical Operator/1 -> IGBT/Diode/1
  Voltage Measurement/1 -> VC/1
  Logical Operator1/1 -> IGBT/Diode1/1
  connections:
  Voltage Measurement/LConn2 -- Series RLC Branch/RConn1 -- IGBT/Diode1/RConn1 -- V-/RConn1
  IGBT/Diode/RConn1 -- IGBT/Diode1/LConn1 -- V+/RConn1
  IGBT/Diode/LConn1 -- Series RLC Branch/LConn1 -- Voltage Measurement/LConn1

== system MMC_Rectifier_NLM_2018/MMC  Rectifier/MMC1/MMC11 ==
  PWM : Inport
  IGBT/Diode : spsIGBTDiodeLib/IGBT//Diode  Ron=1e-3  Rs=1e5  Cs=inf  Measurements=off
  IGBT/Diode1 : spsIGBTDiodeLib/IGBT//Diode  Ron=1e-3  Rs=1e5  Cs=inf  Measurements=off
  Logical Operator : Logic  Inputs=1  AllPortsSameDT=off  OutDataTypeStr=boolean
  Logical Operator1 : Logic  Operator=NOT  Inputs=1  AllPortsSameDT=off  OutDataTypeStr=boolean
  Series RLC Branch : spsSeriesRLCBranchLib/Series RLC Branch  LConnTagsString=__new0  RConnTagsString=__new0  BranchType=C  Resistance=1  Inductance=1e-3  SetiL0=off  InitialCurrent=0  Capacitance=C0  Setx0=on  InitialVoltage=V0  Measurements=None
  Voltage Measurement : spsVoltageMeasurementLib/Voltage Measurement  PhasorSimulation=off  OutputType=Complex  PSBequivalent=0
  V+ : PMIOPort  Side=Left
  V- : PMIOPort  Port=2  Side=Left
  VC : Outport
  wires:
  Logical Operator1/1 -> IGBT/Diode1/1
  Voltage Measurement/1 -> VC/1
  Logical Operator/1 -> IGBT/Diode/1
  PWM/1 -> Logical Operator/1, Logical Operator1/1
  connections:
  Voltage Measurement/LConn1 -- Series RLC Branch/LConn1 -- IGBT/Diode/LConn1
  V+/RConn1 -- IGBT/Diode1/LConn1 -- IGBT/Diode/RConn1
  V-/RConn1 -- IGBT/Diode1/RConn1 -- Series RLC Branch/RConn1 -- Voltage Measurement/LConn2

== system MMC_Rectifier_NLM_2018/MMC  Rectifier/MMC1/MMC12 ==
  PWM : Inport
  IGBT/Diode : spsIGBTDiodeLib/IGBT//Diode  Ron=1e-3  Rs=1e5  Cs=inf  Measurements=off
  IGBT/Diode1 : spsIGBTDiodeLib/IGBT//Diode  Ron=1e-3  Rs=1e5  Cs=inf  Measurements=off
  Logical Operator : Logic  Inputs=1  AllPortsSameDT=off  OutDataTypeStr=boolean
  Logical Operator1 : Logic  Operator=NOT  Inputs=1  AllPortsSameDT=off  OutDataTypeStr=boolean
  Series RLC Branch : spsSeriesRLCBranchLib/Series RLC Branch  LConnTagsString=__new0  RConnTagsString=__new0  BranchType=C  Resistance=1  Inductance=1e-3  SetiL0=off  InitialCurrent=0  Capacitance=C0  Setx0=on  InitialVoltage=V0  Measurements=None
  Voltage Measurement : spsVoltageMeasurementLib/Voltage Measurement  PhasorSimulation=off  OutputType=Complex  PSBequivalent=0
  V+ : PMIOPort  Side=Left
  V- : PMIOPort  Port=2  Side=Left
  VC : Outport
  wires:
  Logical Operator1/1 -> IGBT/Diode1/1
  Voltage Measurement/1 -> VC/1
  Logical Operator/1 -> IGBT/Diode/1
  PWM/1 -> Logical Operator/1, Logical Operator1/1
  connections:
  Voltage Measurement/LConn1 -- Series RLC Branch/LConn1 -- IGBT/Diode/LConn1
  V+/RConn1 -- IGBT/Diode1/LConn1 -- IGBT/Diode/RConn1
  V-/RConn1 -- IGBT/Diode1/RConn1 -- Series RLC Branch/RConn1 -- Voltage Measurement/LConn2

== system MMC_Rectifier_NLM_2018/MMC  Rectifier/MMC1/MMC13 ==
  PWM : Inport
  IGBT/Diode : spsIGBTDiodeLib/IGBT//Diode  Ron=1e-3  Rs=1e5  Cs=inf  Measurements=off
  IGBT/Diode1 : spsIGBTDiodeLib/IGBT//Diode  Ron=1e-3  Rs=1e5  Cs=inf  Measurements=off
  Logical Operator : Logic  Inputs=1  AllPortsSameDT=off  OutDataTypeStr=boolean
  Logical Operator1 : Logic  Operator=NOT  Inputs=1  AllPortsSameDT=off  OutDataTypeStr=boolean
  Series RLC Branch : spsSeriesRLCBranchLib/Series RLC Branch  LConnTagsString=__new0  RConnTagsString=__new0  BranchType=C  Resistance=1  Inductance=1e-3  SetiL0=off  InitialCurrent=0  Capacitance=C0  Setx0=on  InitialVoltage=V0  Measurements=None
  Voltage Measurement : spsVoltageMeasurementLib/Voltage Measurement  PhasorSimulation=off  OutputType=Complex  PSBequivalent=0
  V+ : PMIOPort  Side=Left
  V- : PMIOPort  Port=2  Side=Left
  VC : Outport
  wires:
  PWM/1 -> Logical Operator1/1, Logical Operator/1
  Logical Operator/1 -> IGBT/Diode/1
  Voltage Measurement/1 -> VC/1
  Logical Operator1/1 -> IGBT/Diode1/1
  connections:
  Voltage Measurement/LConn2 -- Series RLC Branch/RConn1 -- IGBT/Diode1/RConn1 -- V-/RConn1
  IGBT/Diode/RConn1 -- IGBT/Diode1/LConn1 -- V+/RConn1
  IGBT/Diode/LConn1 -- Series RLC Branch/LConn1 -- Voltage Measurement/LConn1

== system MMC_Rectifier_NLM_2018/MMC  Rectifier/MMC1/MMC14 ==
  PWM : Inport
  IGBT/Diode : spsIGBTDiodeLib/IGBT//Diode  Ron=1e-3  Rs=1e5  Cs=inf  Measurements=off
  IGBT/Diode1 : spsIGBTDiodeLib/IGBT//Diode  Ron=1e-3  Rs=1e5  Cs=inf  Measurements=off
  Logical Operator : Logic  Inputs=1  AllPortsSameDT=off  OutDataTypeStr=boolean
  Logical Operator1 : Logic  Operator=NOT  Inputs=1  AllPortsSameDT=off  OutDataTypeStr=boolean
  Series RLC Branch : spsSeriesRLCBranchLib/Series RLC Branch  LConnTagsString=__new0  RConnTagsString=__new0  BranchType=C  Resistance=1  Inductance=1e-3  SetiL0=off  InitialCurrent=0  Capacitance=C0  Setx0=on  InitialVoltage=V0  Measurements=None
  Voltage Measurement : spsVoltageMeasurementLib/Voltage Measurement  PhasorSimulation=off  OutputType=Complex  PSBequivalent=0
  V+ : PMIOPort  Side=Left
  V- : PMIOPort  Port=2  Side=Left
  VC : Outport
  wires:
  Logical Operator1/1 -> IGBT/Diode1/1
  Voltage Measurement/1 -> VC/1
  Logical Operator/1 -> IGBT/Diode/1
  PWM/1 -> Logical Operator/1, Logical Operator1/1
  connections:
  IGBT/Diode/LConn1 -- Voltage Measurement/LConn1 -- Series RLC Branch/LConn1
  IGBT/Diode/RConn1 -- V+/RConn1 -- IGBT/Diode1/LConn1
  IGBT/Diode1/RConn1 -- V-/RConn1 -- Voltage Measurement/LConn2 -- Series RLC Branch/RConn1

== system MMC_Rectifier_NLM_2018/MMC  Rectifier/MMC1/MMC15 ==
  PWM : Inport
  IGBT/Diode : spsIGBTDiodeLib/IGBT//Diode  Ron=1e-3  Rs=1e5  Cs=inf  Measurements=off
  IGBT/Diode1 : spsIGBTDiodeLib/IGBT//Diode  Ron=1e-3  Rs=1e5  Cs=inf  Measurements=off
  Logical Operator : Logic  Inputs=1  AllPortsSameDT=off  OutDataTypeStr=boolean
  Logical Operator1 : Logic  Operator=NOT  Inputs=1  AllPortsSameDT=off  OutDataTypeStr=boolean
  Series RLC Branch : spsSeriesRLCBranchLib/Series RLC Branch  LConnTagsString=__new0  RConnTagsString=__new0  BranchType=C  Resistance=1  Inductance=1e-3  SetiL0=off  InitialCurrent=0  Capacitance=C0  Setx0=on  InitialVoltage=V0  Measurements=None
  Voltage Measurement : spsVoltageMeasurementLib/Voltage Measurement  PhasorSimulation=off  OutputType=Complex  PSBequivalent=0
  V+ : PMIOPort  Side=Left
  V- : PMIOPort  Port=2  Side=Left
  VC : Outport
  wires:
  PWM/1 -> Logical Operator1/1, Logical Operator/1
  Logical Operator/1 -> IGBT/Diode/1
  Voltage Measurement/1 -> VC/1
  Logical Operator1/1 -> IGBT/Diode1/1
  connections:
  Voltage Measurement/LConn2 -- Series RLC Branch/RConn1 -- IGBT/Diode1/RConn1 -- V-/RConn1
  IGBT/Diode/RConn1 -- IGBT/Diode1/LConn1 -- V+/RConn1
  IGBT/Diode/LConn1 -- Series RLC Branch/LConn1 -- Voltage Measurement/LConn1

== system MMC_Rectifier_NLM_2018/MMC  Rectifier/MMC1/MMC16 ==
  PWM : Inport
  IGBT/Diode : spsIGBTDiodeLib/IGBT//Diode  Ron=1e-3  Rs=1e5  Cs=inf  Measurements=off
  IGBT/Diode1 : spsIGBTDiodeLib/IGBT//Diode  Ron=1e-3  Rs=1e5  Cs=inf  Measurements=off
  Logical Operator : Logic  Inputs=1  AllPortsSameDT=off  OutDataTypeStr=boolean
  Logical Operator1 : Logic  Operator=NOT  Inputs=1  AllPortsSameDT=off  OutDataTypeStr=boolean
  Series RLC Branch : spsSeriesRLCBranchLib/Series RLC Branch  LConnTagsString=__new0  RConnTagsString=__new0  BranchType=C  Resistance=1  Inductance=1e-3  SetiL0=off  InitialCurrent=0  Capacitance=C0  Setx0=on  InitialVoltage=V0  Measurements=None
  Voltage Measurement : spsVoltageMeasurementLib/Voltage Measurement  PhasorSimulation=off  OutputType=Complex  PSBequivalent=0
  V+ : PMIOPort  Side=Left
  V- : PMIOPort  Port=2  Side=Left
  VC : Outport
  wires:
  PWM/1 -> Logical Operator1/1, Logical Operator/1
  Logical Operator/1 -> IGBT/Diode/1
  Voltage Measurement/1 -> VC/1
  Logical Operator1/1 -> IGBT/Diode1/1
  connections:
  Voltage Measurement/LConn2 -- Series RLC Branch/RConn1 -- IGBT/Diode1/RConn1 -- V-/RConn1
  IGBT/Diode/RConn1 -- IGBT/Diode1/LConn1 -- V+/RConn1
  IGBT/Diode/LConn1 -- Series RLC Branch/LConn1 -- Voltage Measurement/LConn1

== system MMC_Rectifier_NLM_2018/MMC  Rectifier/MMC1/MMC17 ==
  PWM : Inport
  IGBT/Diode : spsIGBTDiodeLib/IGBT//Diode  Ron=1e-3  Rs=1e5  Cs=inf  Measurements=off
  IGBT/Diode1 : spsIGBTDiodeLib/IGBT//Diode  Ron=1e-3  Rs=1e5  Cs=inf  Measurements=off
  Logical Operator : Logic  Inputs=1  AllPortsSameDT=off  OutDataTypeStr=boolean
  Logical Operator1 : Logic  Operator=NOT  Inputs=1  AllPortsSameDT=off  OutDataTypeStr=boolean
  Series RLC Branch : spsSeriesRLCBranchLib/Series RLC Branch  LConnTagsString=__new0  RConnTagsString=__new0  BranchType=C  Resistance=1  Inductance=1e-3  SetiL0=off  InitialCurrent=0  Capacitance=C0  Setx0=on  InitialVoltage=V0  Measurements=None
  Voltage Measurement : spsVoltageMeasurementLib/Voltage Measurement  PhasorSimulation=off  OutputType=Complex  PSBequivalent=0
  V+ : PMIOPort  Side=Left
  V- : PMIOPort  Port=2  Side=Left
  VC : Outport
  wires:
  Logical Operator1/1 -> IGBT/Diode1/1
  Voltage Measurement/1 -> VC/1
  Logical Operator/1 -> IGBT/Diode/1
  PWM/1 -> Logical Operator/1, Logical Operator1/1
  connections:
  Voltage Measurement/LConn1 -- Series RLC Branch/LConn1 -- IGBT/Diode/LConn1
  V+/RConn1 -- IGBT/Diode1/LConn1 -- IGBT/Diode/RConn1
  V-/RConn1 -- IGBT/Diode1/RConn1 -- Series RLC Branch/RConn1 -- Voltage Measurement/LConn2

== system MMC_Rectifier_NLM_2018/MMC  Rectifier/MMC1/MMC2 ==
  PWM : Inport
  IGBT/Diode : spsIGBTDiodeLib/IGBT//Diode  Ron=1e-3  Rs=1e5  Cs=inf  Measurements=off
  IGBT/Diode1 : spsIGBTDiodeLib/IGBT//Diode  Ron=1e-3  Rs=1e5  Cs=inf  Measurements=off
  Logical Operator : Logic  Inputs=1  AllPortsSameDT=off  OutDataTypeStr=boolean
  Logical Operator1 : Logic  Operator=NOT  Inputs=1  AllPortsSameDT=off  OutDataTypeStr=boolean
  Series RLC Branch : spsSeriesRLCBranchLib/Series RLC Branch  LConnTagsString=__new0  RConnTagsString=__new0  BranchType=C  Resistance=1  Inductance=1e-3  SetiL0=off  InitialCurrent=0  Capacitance=C0  Setx0=on  InitialVoltage=V0  Measurements=None
  Voltage Measurement : spsVoltageMeasurementLib/Voltage Measurement  PhasorSimulation=off  OutputType=Complex  PSBequivalent=0
  V+ : PMIOPort  Side=Left
  V- : PMIOPort  Port=2  Side=Left
  VC : Outport
  wires:
  PWM/1 -> Logical Operator1/1, Logical Operator/1
  Logical Operator/1 -> IGBT/Diode/1
  Voltage Measurement/1 -> VC/1
  Logical Operator1/1 -> IGBT/Diode1/1
  connections:
  Voltage Measurement/LConn2 -- Series RLC Branch/RConn1 -- IGBT/Diode1/RConn1 -- V-/RConn1
  IGBT/Diode/RConn1 -- IGBT/Diode1/LConn1 -- V+/RConn1
  IGBT/Diode/LConn1 -- Series RLC Branch/LConn1 -- Voltage Measurement/LConn1

== system MMC_Rectifier_NLM_2018/MMC  Rectifier/MMC1/MMC3 ==
  PWM : Inport
  IGBT/Diode : spsIGBTDiodeLib/IGBT//Diode  Ron=1e-3  Rs=1e5  Cs=inf  Measurements=off
  IGBT/Diode1 : spsIGBTDiodeLib/IGBT//Diode  Ron=1e-3  Rs=1e5  Cs=inf  Measurements=off
  Logical Operator : Logic  Inputs=1  AllPortsSameDT=off  OutDataTypeStr=boolean
  Logical Operator1 : Logic  Operator=NOT  Inputs=1  AllPortsSameDT=off  OutDataTypeStr=boolean
  Series RLC Branch : spsSeriesRLCBranchLib/Series RLC Branch  LConnTagsString=__new0  RConnTagsString=__new0  BranchType=C  Resistance=1  Inductance=1e-3  SetiL0=off  InitialCurrent=0  Capacitance=C0  Setx0=on  InitialVoltage=V0  Measurements=None
  Voltage Measurement : spsVoltageMeasurementLib/Voltage Measurement  PhasorSimulation=off  OutputType=Complex  PSBequivalent=0
  V+ : PMIOPort  Side=Left
  V- : PMIOPort  Port=2  Side=Left
  VC : Outport
  wires:
  Logical Operator1/1 -> IGBT/Diode1/1
  Voltage Measurement/1 -> VC/1
  Logical Operator/1 -> IGBT/Diode/1
  PWM/1 -> Logical Operator/1, Logical Operator1/1
  connections:
  Voltage Measurement/LConn1 -- Series RLC Branch/LConn1 -- IGBT/Diode/LConn1
  V+/RConn1 -- IGBT/Diode1/LConn1 -- IGBT/Diode/RConn1
  V-/RConn1 -- IGBT/Diode1/RConn1 -- Series RLC Branch/RConn1 -- Voltage Measurement/LConn2

== system MMC_Rectifier_NLM_2018/MMC  Rectifier/MMC1/MMC4 ==
  PWM : Inport
  IGBT/Diode : spsIGBTDiodeLib/IGBT//Diode  Ron=1e-3  Rs=1e5  Cs=inf  Measurements=off
  IGBT/Diode1 : spsIGBTDiodeLib/IGBT//Diode  Ron=1e-3  Rs=1e5  Cs=inf  Measurements=off
  Logical Operator : Logic  Inputs=1  AllPortsSameDT=off  OutDataTypeStr=boolean
  Logical Operator1 : Logic  Operator=NOT  Inputs=1  AllPortsSameDT=off  OutDataTypeStr=boolean
  Series RLC Branch : spsSeriesRLCBranchLib/Series RLC Branch  LConnTagsString=__new0  RConnTagsString=__new0  BranchType=C  Resistance=1  Inductance=1e-3  SetiL0=off  InitialCurrent=0  Capacitance=C0  Setx0=on  InitialVoltage=V0  Measurements=None
  Voltage Measurement : spsVoltageMeasurementLib/Voltage Measurement  PhasorSimulation=off  OutputType=Complex  PSBequivalent=0
  V+ : PMIOPort  Side=Left
  V- : PMIOPort  Port=2  Side=Left
  VC : Outport
  wires:
  Logical Operator1/1 -> IGBT/Diode1/1
  Voltage Measurement/1 -> VC/1
  Logical Operator/1 -> IGBT/Diode/1
  PWM/1 -> Logical Operator/1, Logical Operator1/1
  connections:
  Voltage Measurement/LConn1 -- Series RLC Branch/LConn1 -- IGBT/Diode/LConn1
  V+/RConn1 -- IGBT/Diode1/LConn1 -- IGBT/Diode/RConn1
  V-/RConn1 -- IGBT/Diode1/RConn1 -- Series RLC Branch/RConn1 -- Voltage Measurement/LConn2

== system MMC_Rectifier_NLM_2018/MMC  Rectifier/MMC1/MMC5 ==
  PWM : Inport
  IGBT/Diode : spsIGBTDiodeLib/IGBT//Diode  Ron=1e-3  Rs=1e5  Cs=inf  Measurements=off
  IGBT/Diode1 : spsIGBTDiodeLib/IGBT//Diode  Ron=1e-3  Rs=1e5  Cs=inf  Measurements=off
  Logical Operator : Logic  Inputs=1  AllPortsSameDT=off  OutDataTypeStr=boolean
  Logical Operator1 : Logic  Operator=NOT  Inputs=1  AllPortsSameDT=off  OutDataTypeStr=boolean
  Series RLC Branch : spsSeriesRLCBranchLib/Series RLC Branch  LConnTagsString=__new0  RConnTagsString=__new0  BranchType=C  Resistance=1  Inductance=1e-3  SetiL0=off  InitialCurrent=0  Capacitance=C0  Setx0=on  InitialVoltage=V0  Measurements=None
  Voltage Measurement : spsVoltageMeasurementLib/Voltage Measurement  PhasorSimulation=off  OutputType=Complex  PSBequivalent=0
  V+ : PMIOPort  Side=Left
  V- : PMIOPort  Port=2  Side=Left
  VC : Outport
  wires:
  PWM/1 -> Logical Operator1/1, Logical Operator/1
  Logical Operator/1 -> IGBT/Diode/1
  Voltage Measurement/1 -> VC/1
  Logical Operator1/1 -> IGBT/Diode1/1
  connections:
  Voltage Measurement/LConn2 -- Series RLC Branch/RConn1 -- IGBT/Diode1/RConn1 -- V-/RConn1
  IGBT/Diode/RConn1 -- IGBT/Diode1/LConn1 -- V+/RConn1
  IGBT/Diode/LConn1 -- Series RLC Branch/LConn1 -- Voltage Measurement/LConn1

== system MMC_Rectifier_NLM_2018/MMC  Rectifier/MMC1/MMC6 ==
  PWM : Inport
  IGBT/Diode : spsIGBTDiodeLib/IGBT//Diode  Ron=1e-3  Rs=1e5  Cs=inf  Measurements=off
  IGBT/Diode1 : spsIGBTDiodeLib/IGBT//Diode  Ron=1e-3  Rs=1e5  Cs=inf  Measurements=off
  Logical Operator : Logic  Inputs=1  AllPortsSameDT=off  OutDataTypeStr=boolean
  Logical Operator1 : Logic  Operator=NOT  Inputs=1  AllPortsSameDT=off  OutDataTypeStr=boolean
  Series RLC Branch : spsSeriesRLCBranchLib/Series RLC Branch  LConnTagsString=__new0  RConnTagsString=__new0  BranchType=C  Resistance=1  Inductance=1e-3  SetiL0=off  InitialCurrent=0  Capacitance=C0  Setx0=on  InitialVoltage=V0  Measurements=None
  Voltage Measurement : spsVoltageMeasurementLib/Voltage Measurement  PhasorSimulation=off  OutputType=Complex  PSBequivalent=0
  V+ : PMIOPort  Side=Left
  V- : PMIOPort  Port=2  Side=Left
  VC : Outport
  wires:
  PWM/1 -> Logical Operator1/1, Logical Operator/1
  Logical Operator/1 -> IGBT/Diode/1
  Voltage Measurement/1 -> VC/1
  Logical Operator1/1 -> IGBT/Diode1/1
  connections:
  Series RLC Branch/RConn1 -- Voltage Measurement/LConn2 -- V-/RConn1 -- IGBT/Diode1/RConn1
  IGBT/Diode1/LConn1 -- V+/RConn1 -- IGBT/Diode/RConn1
  Series RLC Branch/LConn1 -- Voltage Measurement/LConn1 -- IGBT/Diode/LConn1
